simulink model "quarter_car"  (R2025b)
settings: Solver=ode45  StartTime=0.0  StopTime=p.stopTime  MaxStep=p.sampleTime  RelTol=1e-8  AbsTol=1e-10
model workspace (MAT data in the model file):
  A = [0  1  0  0; -56.25  -3.75  56.25  3.75; 0  0  0  1; 400  26.6666666667  -4511.11111111  -26.6666666667]
  Br = [0; 0; 0; 4111.11111111]
  Bu = [0; 0.003125; 0; -0.0222222222222]
  K = [-8856.72818689 987.446391735 12981.1523531 752.758861065]
  p.sprungMass = 320
  p.unsprungMass = 45
  p.suspensionStiffness = 18000
  p.suspensionDamping = 1200
  p.tireStiffness = 185000
  p.skyhookDamping = 2200
  p.forceLimit = 1200
  p.bumpHeight = 0.02
  p.bumpTime = 0.2
  p.bumpDuration = 0.25
  p.sampleTime = 0.001
  p.stopTime = 3.015
  roadInput = timeseries
  roadInput.Name = 'unnamed'
  roadInput.DataInfo = tsdata.datametadata
  roadInput.DataInfo.Interpolation = tsdata.interpolation
  roadInput.DataInfo.Interpolation.Fhandle : function handle (value not decoded)
  roadInput.DataInfo.Interpolation.Name = 'linear'
  roadInput.TimeInfo = tsdata.timemetadata
  roadInput.TimeInfo.Length = 3016
  roadInput.TimeInfo.DuplicateTimes = 0
  roadInput.TimeInfo.Time_ = [0 0.001 0.002 0.003 0.004 0.005 0.006 0.007 0.008 0.009 0.01 0.011 ... (3016 elements, 3016x1)]
  roadInput.TimeInfo.Initialized = 1
  roadInput.QualityInfo = tsdata.qualmetadata
  roadInput.Data_ = [0 0 0 0 0 0 0 0 0 0 0 0 ... (3016 elements, 3016x1)]
values from neighbouring files (symbols this model uses):
  p = project_parameters()    [run_demo.m]
settings Model: Creator=LENOVO  LastModifiedBy=LENOVO

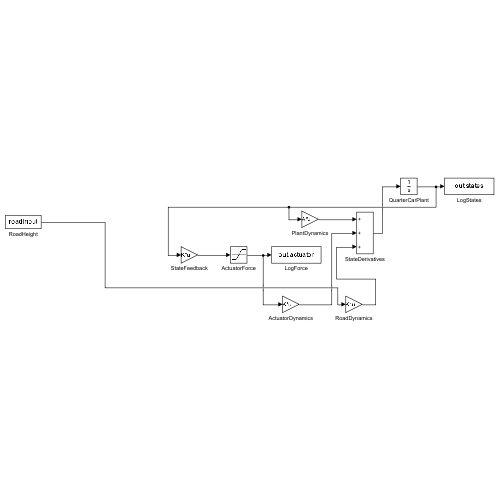
[thumbnail: Simulink's stored preview of the top-level diagram]
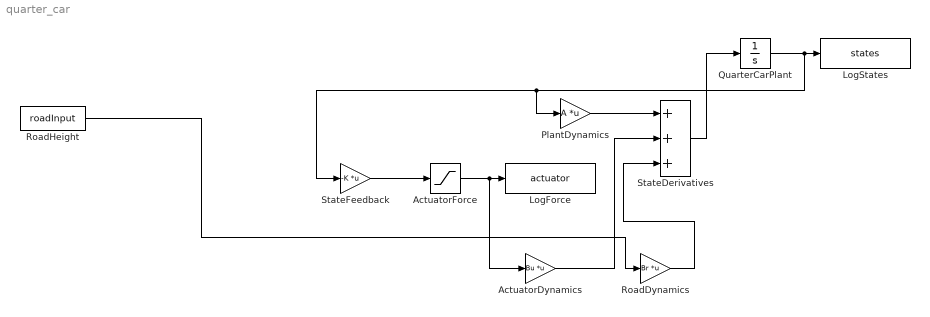
== system quarter_car ==
  ActuatorDynamics : Gain  Gain=Bu  Multiplication=Matrix(K*u)
  ActuatorForce : Saturate  UpperLimit=p.forceLimit  LowerLimit=-p.forceLimit
  LogForce : ToWorkspace  VariableName=actuator  SaveFormat=Timeseries  SampleTime=-1
  LogStates : ToWorkspace  VariableName=states  SaveFormat=Timeseries  SampleTime=-1
  PlantDynamics : Gain  Gain=A  Multiplication=Matrix(K*u)
  QuarterCarPlant : Integrator  InitialCondition=zeros(4,1)
  RoadDynamics : Gain  Gain=Br  Multiplication=Matrix(K*u)
  RoadHeight : FromWorkspace  VariableName=roadInput
  StateDerivatives : Sum  Inputs=+++
  StateFeedback : Gain  Gain=-K  Multiplication=Matrix(K*u)
  wires:
  StateFeedback/1 -> ActuatorForce/1
  StateDerivatives/1 -> QuarterCarPlant/1
  RoadDynamics/1 -> StateDerivatives/3
  ActuatorDynamics/1 -> StateDerivatives/2
  PlantDynamics/1 -> StateDerivatives/1
  RoadHeight/1 -> RoadDynamics/1
  QuarterCarPlant/1 -> PlantDynamics/1, StateFeedback/1, LogStates/1
  ActuatorForce/1 -> ActuatorDynamics/1, LogForce/1
